simulink model "aero2_hardware_cascade_offline_R2021a"  (R2021a)
settings: Solver=ode1  StartTime=0.0  StopTime=60  FixedStep=0.002  RelTol=1e-3
model workspace (MAT data in the model file):
  Dq = 2.25
  Kaw = 20
  Kff = 1
  Ki = 1.84164606325
  Kp = 0.216370391856
  Kq = 2.25
  ReferenceRate = [0 0.002 0.004 0.006 0.008 0.01 0.012 0.014 0.016 0.018 0.02 0.022 ... (90003 elements, 30001x3)]
  Ts = 0.002
  U_h : timeseries (value not decoded)
  U_v : timeseries (value not decoded)
  X0 = [0; 0; 0; 0]
  meas_on = 0
undefined symbols (not defined in the file): DiscIntNeverNeededParam
(part 2 of 2)

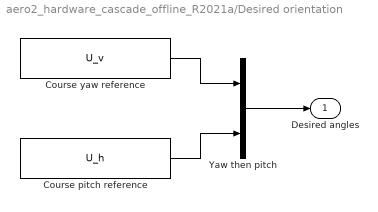
== system aero2_hardware_cascade_offline_R2021a/Desired orientation ==
  Course pitch reference : FromWorkspace  VariableName=U_h  OutputAfterFinalValue=Holding final value
  Course yaw reference : FromWorkspace  VariableName=U_v  OutputAfterFinalValue=Holding final value
  Yaw then pitch : Mux  Inputs=2
  Desired angles : Outport
  wires:
  Course yaw reference/1 -> Yaw then pitch/1
  Course pitch reference/1 -> Yaw then pitch/2
  Yaw then pitch/1 -> Desired angles/1

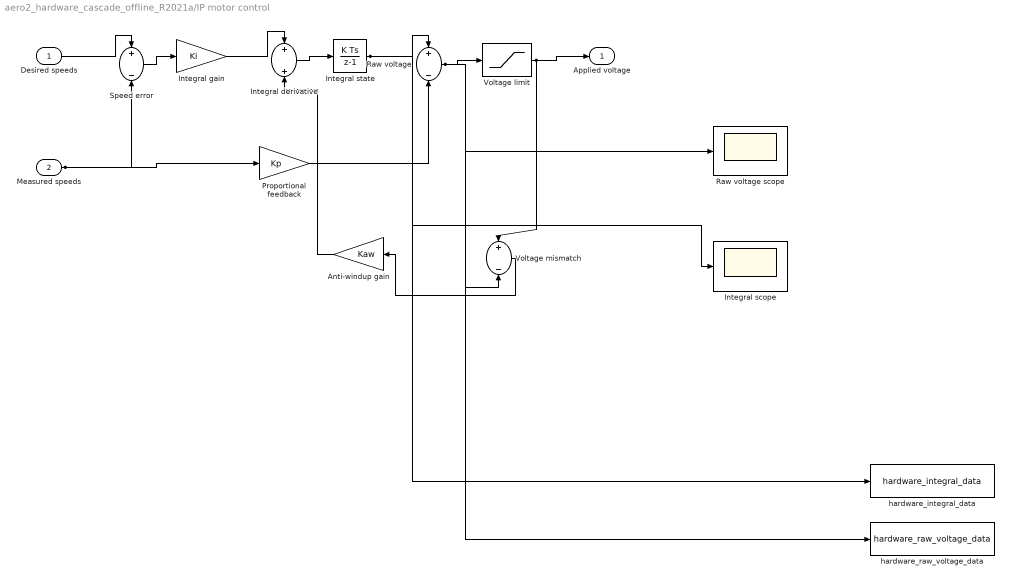
== system aero2_hardware_cascade_offline_R2021a/IP motor control ==
  Desired speeds : Inport
  Measured speeds : Inport  Port=2
  Anti-windup gain : Gain  Gain=Kaw
  Integral derivative : Sum
  Integral gain : Gain  Gain=Ki
  Integral scope : Scope
  Integral state : DiscreteIntegrator  InitialCondition=[0;0]  SampleTime=Ts  ICPrevOutput=DiscIntNeverNeededParam  ICPrevScaledInput=DiscIntNeverNeededParam
  Proportional feedback : Gain  Gain=Kp
  Raw voltage : Sum  Inputs=+-
  Raw voltage scope : Scope
  Speed error : Sum  Inputs=+-
  Voltage limit : Saturate  UpperLimit=24  LowerLimit=-24
  Voltage mismatch : Sum  Inputs=+-
  hardware_integral_data : ToWorkspace  VariableName=hardware_integral_data  SaveFormat=Timeseries  SampleTime=-1
  hardware_raw_voltage_data : ToWorkspace  VariableName=hardware_raw_voltage_data  SaveFormat=Timeseries  SampleTime=-1
  Applied voltage : Outport
  wires:
  Desired speeds/1 -> Speed error/1
  Measured speeds/1 -> Speed error/2, Proportional feedback/1
  Speed error/1 -> Integral gain/1
  Integral gain/1 -> Integral derivative/1
  Proportional feedback/1 -> Raw voltage/2
  Raw voltage/1 -> Voltage limit/1, Voltage mismatch/2, Raw voltage scope/1, hardware_raw_voltage_data/1
  Voltage limit/1 -> Applied voltage/1, Voltage mismatch/1
  Voltage mismatch/1 -> Anti-windup gain/1
  Anti-windup gain/1 -> Integral derivative/2
  Integral derivative/1 -> Integral state/1
  Integral state/1 -> Raw voltage/1, Integral scope/1, hardware_integral_data/1

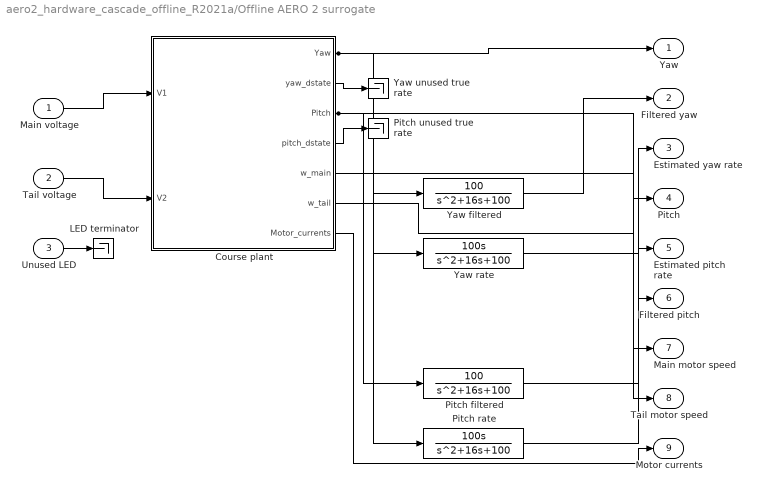
== system aero2_hardware_cascade_offline_R2021a/Offline AERO 2 surrogate ==
  Main voltage : Inport
  Tail voltage : Inport  Port=2
  Unused LED : Inport  Port=3
  Course plant : Subsystem  mask{meas=meas_on}
      mask prompts: meas "Measurement effects (1 = encoder quantization + sensor noise, 0 = ideal)"
      mask help: Simplified twin-rotor model (eq. (simp) of twin_rotor_FL_merged.tex) with DC-motor rotor dynamics. Inputs: V1 main-rotor voltage, V2 tail-rotor voltage [V]. Outputs: same signals as the QUARC interface of lin_feedback_v1.slx, continuous (no zero-order holds; sensor noise generated at Ts).
  LED terminator : Terminator
  Pitch filtered : TransferFcn  Numerator=100  Denominator=[1 16 100]
  Pitch rate : TransferFcn  Numerator=[100 0]  Denominator=[1 16 100]
  Pitch unused true rate : Terminator
  Yaw filtered : TransferFcn  Numerator=100  Denominator=[1 16 100]
  Yaw rate : TransferFcn  Numerator=[100 0]  Denominator=[1 16 100]
  Yaw unused true rate : Terminator
  Yaw : Outport
  Filtered yaw : Outport  Port=2
  Estimated yaw rate : Outport  Port=3
  Pitch : Outport  Port=4
  Estimated pitch rate : Outport  Port=5
  Filtered pitch : Outport  Port=6
  Main motor speed : Outport  Port=7
  Tail motor speed : Outport  Port=8
  Motor currents : Outport  Port=9
  wires:
  Main voltage/1 -> Course plant/1(V1)
  Tail voltage/1 -> Course plant/2(V2)
  Unused LED/1 -> LED terminator/1
  Course plant/1(Yaw) -> Yaw filtered/1, Yaw rate/1, Yaw/1
  Course plant/2(yaw_dstate) -> Yaw unused true rate/1
  Course plant/3(Pitch) -> Pitch filtered/1, Pitch rate/1, Pitch/1
  Course plant/4(pitch_dstate) -> Pitch unused true rate/1
  Yaw filtered/1 -> Filtered yaw/1
  Yaw rate/1 -> Estimated yaw rate/1
  Pitch rate/1 -> Estimated pitch rate/1
  Pitch filtered/1 -> Filtered pitch/1
  Course plant/5(w_main) -> Main motor speed/1
  Course plant/6(w_tail) -> Tail motor speed/1
  Course plant/7(Motor_currents) -> Motor currents/1

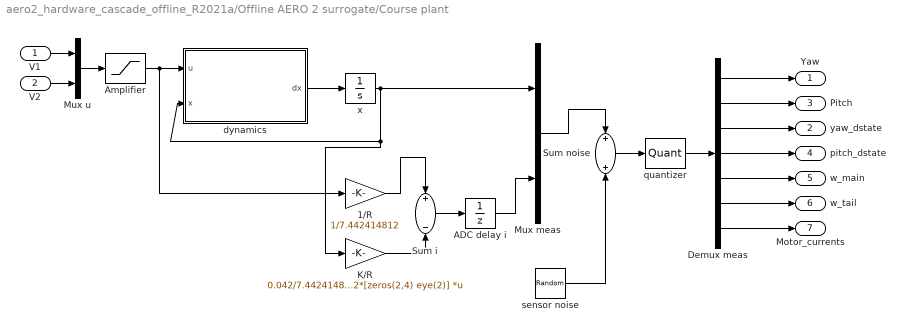
== system aero2_hardware_cascade_offline_R2021a/Offline AERO 2 surrogate/Course plant ==
  V1 : Inport
  V2 : Inport  Port=2
  1/R : Gain  Gain=1/7.442414812
  ADC delay i : UnitDelay  InitialCondition=[0;0]  SampleTime=0.002
  Amplifier : Saturate  UpperLimit=24  LowerLimit=-24
  Demux meas : Demux  Outputs=[1 1 1 1 1 1 2]
  K/R : Gain  Gain=0.042/7.442414812*[zeros(2,4) eye(2)]  Multiplication=Matrix(K*u)
  Mux meas : Mux  Inputs=[6 2]
  Mux u : Mux  Inputs=2
  Sum i : Sum  Inputs=+-
  Sum noise : Sum
  dynamics : MATLAB Function  TreatAsAtomicUnit=on
  quantizer : Quantizer  QuantizationInterval=max((meas)*[0.0015339807878856412;0.0030679615757712823;0.001;0.001;0.050000000000000003;0.050000000000000003;0.001;0.001], 1e-12)
  sensor noise : RandomNumber  Mean=zeros(8,1)  Variance=((meas)*[0.0005;0.0005;0.005;0.005;0.3;0.3;0.01;0.01]).^2  Seed=[61027;18839;4421;30893;23341;7781;51117;9013]  SampleTime=0.002
  x : Integrator  InitialCondition=zeros(6,1)
  Yaw : Outport
  yaw_dstate : Outport  Port=2
  Pitch : Outport  Port=3
  pitch_dstate : Outport  Port=4
  w_main : Outport  Port=5
  w_tail : Outport  Port=6
  Motor_currents : Outport  Port=7
  wires:
  Demux meas/7 -> Motor_currents/1
  Demux meas/6 -> w_tail/1
  Demux meas/5 -> w_main/1
  Demux meas/4 -> pitch_dstate/1
  Demux meas/2 -> Pitch/1
  Demux meas/3 -> yaw_dstate/1
  Demux meas/1 -> Yaw/1
  quantizer/1 -> Demux meas/1
  Sum noise/1 -> quantizer/1
  sensor noise/1 -> Sum noise/2
  Mux meas/1 -> Sum noise/1
  ADC delay i/1 -> Mux meas/2
  Sum i/1 -> ADC delay i/1
  K/R/1 -> Sum i/2
  1/R/1 -> Sum i/1
  x/1 -> K/R/1, dynamics/2(x), Mux meas/1
  dynamics/1(dx) -> x/1
  Amplifier/1 -> 1/R/1, dynamics/1(u)
  Mux u/1 -> Amplifier/1
  V2/1 -> Mux u/2
  V1/1 -> Mux u/1

== matlab function aero2_hardware_cascade_offline_R2021a/Offline AERO 2 surrogate/Course plant/dynamics ==
  data: u input; dx output; x input
function dx = fcn(u, x)
%% Simplified twin-rotor model of aero2_model.pdf (2-DOF body + first-order motors)
p = struct('Jph', 0.64070000000000005, ...
    'jph', 0.01, ...
    'Jth', 0.71640000000000004, ...
    'G', 0.025399999999999999, ...
    'kT', 4.2486999999999997e-06, ...
    'kF', 2.5525999999999999e-05, ...
    'L', 0.16700000000000001, ...
    'Cor', 0.63070000000000004, ...
    'Dph', 0, ...
    'Dth', 0, ...
    'aw', 5.7800000000000002, ...
    'bw', 96.531999999999996);
dx = tr_simp_dyn(x, u, p);
end

function dx = tr_simp_dyn(x, u, p)
%TR_SIMP_DYN  Simplified twin-rotor model with voltage inputs (aero2_model.pdf).
%   Body: reduced 2-DOF model, eq. (simp)
%     Mq(th) [ddpsi; ddth] + cq + Bq dq + gq = Gamma(th) [wm|wm|; wt|wt|]
%   with cq = [-Cor sin(2th) dth dpsi; 1/2 Cor sin(2th) dpsi^2]
%   (no gyroscopic coupling, no motor reaction channel, s_m=+1, s_t=-1).
%   Rotors: first-order motor model of the hand-out
%     dw = -aw w + bw v
%   State x = [psi, theta, dpsi, dtheta, wm, wt], input u = [Um, Ut].
%   p: Jph jph Jth Dph Dth Cor L G kF kT aw bw (psim of tr_instructor_params).

    th = x(2);  dps = x(3);  dth = x(4);
    c = cos(th);  s = sin(th);
    tau = [x(5)*abs(x(5)); x(6)*abs(x(6))];

    Ms  = [p.Jph*c^2 + p.jph*s^2, 0; 0, p.Jth];
    Cs  = [-p.Cor*sin(2*th)*dth*dps; 0.5*p.Cor*sin(2*th)*dps^2];
    Ds  = [p.Dph*dps; p.Dth*dth];
    Gs  = [0; p.G*s];
    Gam = [c 0; 0 1]*[-p.kT, p.L*p.kF; p.L*p.kF, p.kT];
    ddq = Ms\(Gam*tau - Cs - Ds - Gs);

    dw  = -p.aw*x(5:6) + p.bw*u(:);
    dx  = [x(3:4); ddq; dw];
end

== matlab function aero2_hardware_cascade_offline_R2021a/Mechanical inverse ==
  data: q input; omegaDesired output; dq input; a input
function omegaDesired = aero2_feedback_linearization(q, dq, a)
%AERO2_FEEDBACK_LINEARIZATION Ideal motor tracking: choose omega for q_ddot=a.
% The signed square root is defined at zero but has no finite derivative there.
p = aero2_mechanical_parameters;
assert(abs(q(2)) <= p.pitchLimit, 'Pitch envelope exceeded (limit 60 deg).');
[M, c, g, Gamma] = aero2_mechanical_terms(q, dq);
s = Gamma\(M*a+c+g);
omegaDesired = sign(s).*sqrt(abs(s));
end

function [M, c, g, Gamma] = aero2_mechanical_terms(q, dq)
%AERO2_MECHANICAL_TERMS M*q_ddot+c+g=Gamma*(omega.*abs(omega)).
% Signal order: q=[yaw;pitch], dq=[yaw rate;pitch rate], omega=[main;tail].
p = aero2_mechanical_parameters;
theta = q(2);
cor = p.Jyaw-p.jyaw;
M = [p.Jyaw*cos(theta)^2+p.jyaw*sin(theta)^2, 0; 0, p.Jpitch];
c = [-cor*sin(2*theta)*dq(2)*dq(1); ...
    0.5*cor*sin(2*theta)*dq(1)^2];
g = [0; p.gravity*sin(theta)];
Gamma = [cos(theta), 0; 0, 1]*[-p.kt, p.lever*p.kf; p.lever*p.kf, p.kt];
end

function p = aero2_mechanical_parameters
%AERO2_MECHANICAL_PARAMETERS Simplified course model, Part II, pages 4-5.
p.Jyaw = 0.6407;
p.jyaw = 0.01;
p.Jpitch = 0.7164;
p.gravity = 0.0254;
p.kt = 4.2487e-6;
p.kf = 2.5526e-5;
p.lever = 0.167;
p.pitchLimit = pi/3; % Simulation envelope, not an approved hardware limit.
p.initialState = [0.1; 0.2; -0.05; 0.04]; % [yaw; pitch; yaw rate; pitch rate].
p.acceleration = [0.15; -0.1];
p.step = 0.002;
end
